simulink model "Kirov_physics"  (R2024b)
settings: Solver=FixedStepDiscrete  StartTime=0.0  StopTime=inf  FixedStep=dt  RelTol=1e-3
undefined symbols (not defined in the file): accel_O, airspeed_bp, alpha_B, alpha_bp, alphaFull, alphaOff, b, battery_capacity_bp, battery_current_bp, battery_initial_capacity_mAh, battery_voltage_table, beta_bp, betaFull, betaOff, brake, brakes, c, channels, CLa, Clb, Clp, CLq, Clr, Cma, Cmq, Cnb, Cnp, Cnr, current_table, DiscIntNeverNeededParam, dt, ELEV_bp, elevator, f, flap, flaps, FLAPS_bp, gear, heightFadeStart, heightOff, hgt_0, Inertia_body, Inertia_load, kInduced, L_aileron, L_throttle, LAILE_bp, lat_0, lon_0, M_aile, M_body, M_elev, M_flap, M_front_gear, M_load, M_main_gear, M_prop, M_rudd, M_spoiler, minWingHeight ... (+36)
libraries: sm_lib x673, simulink x58, nesl_utility x51, simulink_extras x24, uavmavlinklib x12, instrumentlib x4, vrlib x3, aerolibfltsims x3, sharedtransform x3, eeGeneralControl x2, aerolibutil x2, AP_Connector x2
(part 3 of 6)

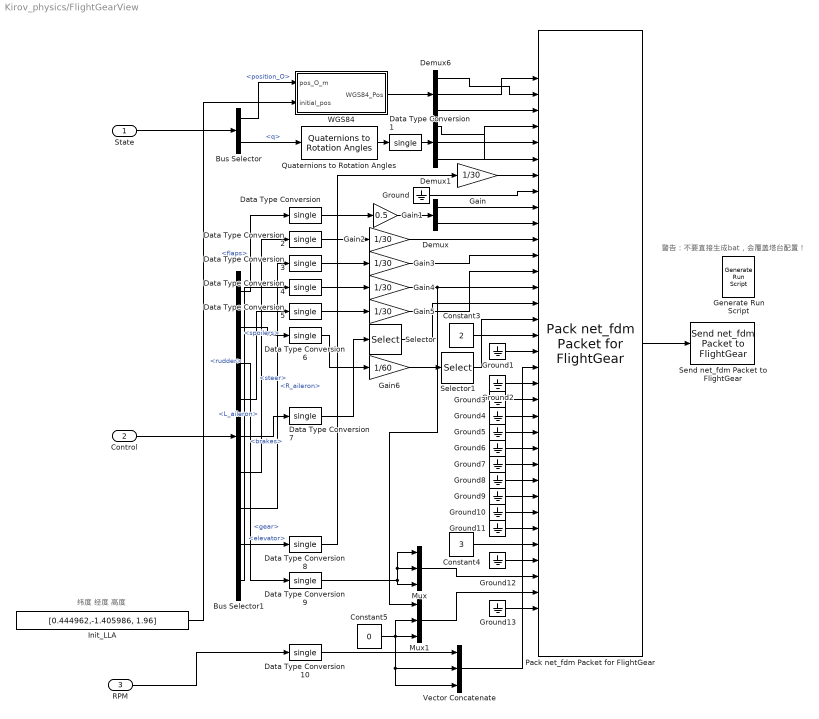
== system Kirov_physics/FlightGearView ==
  note: 警告：不要直接生成bat，会覆盖塔台配置！
  note: 纬度 经度 高度
  State : Inport
  Control : Inport  Port=2
  RPM : Inport  Port=3
  Bus Selector : BusSelector  OutputSignals=position_O,q
  Bus Selector1 : BusSelector  OutputSignals=flaps,spoilers,gear,steer,brakes,L_aileron,R_aileron,elevator,rudder
  Constant3 : Constant  Value=2  OutDataTypeStr=uint32
  Constant4 : Constant  Value=3  OutDataTypeStr=uint32
  Constant5 : Constant  Value=0  OutDataTypeStr=single
  Data Type Conversion{,1..10} (11 alike) : DataTypeConversion  OutDataTypeStr=single  SaturateOnIntegerOverflow=off  RndMeth=Floor
  Demux : Demux  Outputs=2
  Demux1 : Demux  Outputs=3
  Demux6 : Demux  Outputs=3
  Gain{,2..5} (5 alike) : Gain  Gain=1/30
  Gain1 : Gain  Gain=0.5
  Gain6 : Gain  Gain=1/60
  Generate Run Script : aerolibfltsims/Generate Run Script  Architecture=Win64  dataFlow=Send  GeometryModelName=Kirov  AirportId=X51  RunwayId=36  InitialAltitude=2  InitialHeading=0  OffsetDistance=0  OffsetAzimuth=0  InstallScenery=off  DisableShaders=off  OriginAddress=127.0.0.1  DestinationPort=5502  OriginPort=5505  LocalAddress=127.0.0.1  OutputFileName=runfg.bat  FlightGearBaseDirectory=E:\FlightGear 2024.1\
  Ground{,1..13} (14 alike) : Ground
  Init_LLA : Constant  Value=[0.444962,-1.405986, 1.96]  OutDataTypeStr=double
  Mux : Mux  Inputs=3
  Mux1 : Mux  Inputs=3
  Pack net_fdm Packet for FlightGear : aerolibfltsims/Pack net_fdm Packet for FlightGear  FlightGearVersion=v2019.1  ShowPositionAttitudeInputs=on  ShowVelocityAccelerationInputs=off  ShowControlSurfacePositionInputs=on  ShowEngineFuelInputs=on  ShowLandingGearInputs=on  ShowEnvironmentInputs=off  SampleTime=1/100  packetVersion=24
  Quaternions to Rotation Angles : sharedtransform/Quaternions to Rotation Angles  rotationOrder=ZYX  aMode=aMode
  Selector : Selector  InputPortWidth=2  IndexOptions=Index vector (dialog)  Indices=[1]  OutputSizes=1
  Selector1 : Selector  InputPortWidth=2  IndexOptions=Index vector (dialog)  Indices=[1]  OutputSizes=1
  Send net_fdm Packet to FlightGear : aerolibfltsims/Send net_fdm Packet to FlightGear  DestinationIpAddress=127.0.0.1  DestinationPort=5502  LocalIpPort=-1  varLen=off  SampleTime=1/100
  Vector Concatenate : Concatenate  NumInputs=3
  WGS84 : Subsystem
  wires:
  Data Type Conversion2/1 -> Gain2/1
  Quaternions to Rotation Angles/1 -> Data Type Conversion1/1
  State/1 -> Bus Selector/1
  Demux6/2 -> Pack net_fdm Packet for FlightGear/1
  Data Type Conversion1/1 -> Demux1/1
  Bus Selector1/7 -> Data Type Conversion3/1  "<R_aileron>"
  Data Type Conversion9/1 -> Mux/1, Mux/2, Mux/3
  Data Type Conversion5/1 -> Gain5/1
  Demux1/3 -> Pack net_fdm Packet for FlightGear/4
  Data Type Conversion4/1 -> Gain4/1
  Selector1/1 -> Pack net_fdm Packet for FlightGear/16
  Demux/1 -> Pack net_fdm Packet for FlightGear/9
  Gain4/1 -> Mux1/1, Pack net_fdm Packet for FlightGear/13
  Constant5/1 -> Mux1/3, Mux1/2, Vector Concatenate/2, Vector Concatenate/3
  Bus Selector1/4 -> Data Type Conversion5/1  "<steer>"
  Gain1/1 -> Demux/1
  Constant4/1 -> Pack net_fdm Packet for FlightGear/30
  Bus Selector1/8 -> Data Type Conversion8/1  "<elevator>"
  Ground/1 -> Pack net_fdm Packet for FlightGear/8
  Pack net_fdm Packet for FlightGear/1 -> Send net_fdm Packet to FlightGear/1
  Bus Selector1/9 -> Data Type Conversion4/1  "<rudder>"
  Demux1/2 -> Pack net_fdm Packet for FlightGear/5
  Vector Concatenate/1 -> Pack net_fdm Packet for FlightGear/19
  Constant3/1 -> Pack net_fdm Packet for FlightGear/17
  Ground6/1 -> Pack net_fdm Packet for FlightGear/24
  Ground11/1 -> Pack net_fdm Packet for FlightGear/29
  Ground7/1 -> Pack net_fdm Packet for FlightGear/25
  Mux1/1 -> Pack net_fdm Packet for FlightGear/33
  Ground9/1 -> Pack net_fdm Packet for FlightGear/27
  Ground8/1 -> Pack net_fdm Packet for FlightGear/26
  Bus Selector1/5 -> Data Type Conversion7/1  "<brakes>"
  Mux/1 -> Pack net_fdm Packet for FlightGear/32
  Bus Selector/1 -> WGS84/1(pos_O_m)  "<position_O>"
  Bus Selector/2 -> Quaternions to Rotation Angles/1  "<q>"
  Ground2/1 -> Pack net_fdm Packet for FlightGear/20
  WGS84/1(WGS84_Pos) -> Demux6/1
  Ground1/1 -> Pack net_fdm Packet for FlightGear/18
  Selector/1 -> Pack net_fdm Packet for FlightGear/15
  Data Type Conversion6/1 -> Gain6/1
  Gain3/1 -> Pack net_fdm Packet for FlightGear/12
  Ground5/1 -> Pack net_fdm Packet for FlightGear/23
  Bus Selector1/3 -> Data Type Conversion9/1  "<gear>"
  Ground3/1 -> Pack net_fdm Packet for FlightGear/21
  Bus Selector1/2 -> Data Type Conversion6/1  "<spoilers>"
  Demux/2 -> Pack net_fdm Packet for FlightGear/10
  Data Type Conversion3/1 -> Gain3/1
  Data Type Conversion7/1 -> Selector/1
  Ground4/1 -> Pack net_fdm Packet for FlightGear/22
  Ground12/1 -> Pack net_fdm Packet for FlightGear/31
  Data Type Conversion10/1 -> Vector Concatenate/1
  Gain5/1 -> Pack net_fdm Packet for FlightGear/14
  Gain2/1 -> Pack net_fdm Packet for FlightGear/11
  Ground10/1 -> Pack net_fdm Packet for FlightGear/28
  Ground13/1 -> Pack net_fdm Packet for FlightGear/34
  Demux1/1 -> Pack net_fdm Packet for FlightGear/6
  Data Type Conversion8/1 -> Gain/1
  Data Type Conversion/1 -> Gain1/1
  Bus Selector1/6 -> Data Type Conversion2/1  "<L_aileron>"
  Init_LLA/1 -> WGS84/2(initial_pos)
  Demux6/1 -> Pack net_fdm Packet for FlightGear/2
  Gain/1 -> Pack net_fdm Packet for FlightGear/7
  Bus Selector1/1 -> Data Type Conversion/1  "<flaps>"
  Demux6/3 -> Pack net_fdm Packet for FlightGear/3
  Control/1 -> Bus Selector1/1
  RPM/1 -> Data Type Conversion10/1
  Gain6/1 -> Selector1/1

== system Kirov_physics/Power ==
  Current : Inport
  Reset : ResetPort  DisableCoverage=on
  Battery_Voltage_LUT : Lookup_n-D  BreakpointsForDimension1=battery_current_bp  BreakpointsForDimension2=battery_capacity_bp  Table=battery_voltage_table  InterpMethod=Linear Lagrange  ExtrapMethod=Clip  InternalRulePriority=Speed  RndMeth=Simplest
      settings: InputPortMap=u0,u1
  Constant : Constant  Value=0
  Current_Limits : Saturate  UpperLimit=battery_current_bp(end)  LowerLimit=0
  Current_to_mAh_per_s : Gain  Gain=1/3.6
  Discharged_Capacity : DiscreteIntegrator  gainval=1  InitialCondition=battery_initial_capacity_mAh  SampleTime=-1  LimitOutput=on  UpperSaturationLimit=battery_capacity_bp(end)  LowerSaturationLimit=0  ShowSaturationPort=on  ICPrevOutput=DiscIntNeverNeededParam  ICPrevScaledInput=DiscIntNeverNeededParam
  Sum of Elements : Sum  Inputs=+
  Switch : Switch  Criteria=u2 > Threshold  Threshold=0.5  SaturateOnIntegerOverflow=off  InputSameDT=off
  voltage : Outport
  wires:
  Battery_Voltage_LUT/1 -> Switch/3  "V_bat_V"
  Discharged_Capacity/1 -> Battery_Voltage_LUT/2  "Q_dis_mAh"
  Current_to_mAh_per_s/1 -> Discharged_Capacity/1
  Current_Limits/1 -> Current_to_mAh_per_s/1, Battery_Voltage_LUT/1
  Sum of Elements/1 -> Current_Limits/1  "I_bus_A"
  Current/1 -> Sum of Elements/1
  Discharged_Capacity/2 -> Switch/2  "Battery_End"
  Switch/1 -> voltage/1
  Constant/1 -> Switch/1

== system Kirov_physics/Referee ==
  state : Inport
  Add Constant : Bias  Bias=50  SaturateOnIntegerOverflow=off
  Bus Selector : BusSelector  OutputSignals=position_O
  Constant : Constant  Value=2
  Constant1 : Constant  Value=0
  Demux : Demux  Outputs=3
  Gain : Gain  Gain=-1
  Less Than : RelationalOperator  Operator=<  OutDataTypeStr=boolean  RndMeth=Simplest  InputSameDT=off
  Less Than1 : RelationalOperator  Operator=<  OutDataTypeStr=boolean  RndMeth=Simplest  InputSameDT=off
  Less Than2 : RelationalOperator  Operator=>  OutDataTypeStr=boolean  RndMeth=Simplest  InputSameDT=off
  MATLAB Function1 : MATLAB Function  TreatAsAtomicUnit=on
  Manual Switch : ManualSwitch  CurrentSetting=0
  OR : Logic  Operator=OR  AllPortsSameDT=off  OutDataTypeStr=boolean
  Resettable Subsystem : Subsystem  TreatAsAtomicUnit=on
  Safety_Line : Constant  Value=0.5
  Stop Simulation : Stop
  Terminator : Terminator
  wires:
  state/1 -> Bus Selector/1
  Bus Selector/1 -> Demux/1  "<position_O>"
  Demux/1 -> Less Than2/1, Less Than1/1
  Demux/2 -> Less Than/1
  Safety_Line/1 -> Less Than/2
  Demux/3 -> Terminator/1
  Less Than/1 -> MATLAB Function1/1(u)
  Constant/1 -> Add Constant/1
  Less Than1/1 -> OR/1
  Add Constant/1 -> Gain/1, Less Than2/2
  Gain/1 -> Less Than1/2
  Less Than2/1 -> OR/2
  OR/1 -> Resettable Subsystem/1(beep)
  MATLAB Function1/1(y) -> Manual Switch/1
  Manual Switch/1 -> Stop Simulation/1
  Constant1/1 -> Manual Switch/2

== system Kirov_physics/SendState ==
  State : Inport
  Ardupilot : Subsystem  VariantControl=Ardupilot
  Mavlink : Subsystem  VariantControl=Mavlink

== system Kirov_physics/Train_Counter ==
  reset : Inport
  Add2 : Sum
  Minus : Sum  Inputs=+-
  Saturation : Saturate  UpperLimit=1  LowerLimit=0
  Unit Delay2 : UnitDelay  SampleTime=-1  HasFrameUpgradeWarning=on
  Unit Delay3 : UnitDelay  SampleTime=-1  HasFrameUpgradeWarning=on
  count : Outport
  wires:
  Unit Delay3/1 -> Add2/2
  Add2/1 -> count/1, Unit Delay3/1
  Unit Delay2/1 -> Minus/2
  Minus/1 -> Saturation/1
  reset/1 -> Minus/1, Unit Delay2/1
  Saturation/1 -> Add2/1

== system Kirov_physics/wind_NED ==
  wind_ned : Inport
  Bus Assignment : BusAssignment  AssignedSignals=timestamp,V_wind_O
  Constant : Constant  Value=0  OutDataTypeStr=Bus: Environment
  timestamp : Subsystem  mask{sample_time=1000*dt}
      mask prompts: sample_time "sample time (ms)"
  Env : Outport
  wires:
  Bus Assignment/1 -> Env/1
  Constant/1 -> Bus Assignment/1
  wind_ned/1 -> Bus Assignment/3
  timestamp/1(timestamp_ms) -> Bus Assignment/2

== system Kirov_physics/Actuator/Subsystem1 ==
  in : Inport
  Delay : Delay  DelayLengthSource=Input port  InitialConditionSource=Input port
      settings: InputPortMap=u0,p1,p4
  Divide : Product  Inputs=*/
  Round : Rounding  Operator=ceil
  delay_s : Constant  Value=delay_s
  dt_s : Constant  Value=dt
  dynamic_rate_saturation : Subsystem
  rate_limit_1/s : Constant  Value=rate_limit_per_s
  out : Outport
  wires:
  Round/1 -> Delay/2
  Delay/1 -> dynamic_rate_saturation/1(control_in)
  dynamic_rate_saturation/1(control_out) -> out/1  "out"
  in/1 -> Delay/3, Delay/1
  Divide/1 -> Round/1
  delay_s/1 -> Divide/1
  rate_limit_1/s/1 -> dynamic_rate_saturation/2(rate)
  dt_s/1 -> Divide/2

== system Kirov_physics/Actuator/Subsystem2 ==
  in : Inport
  Delay : Delay  DelayLengthSource=Input port  InitialConditionSource=Input port
      settings: InputPortMap=u0,p1,p4
  Divide : Product  Inputs=*/
  Round : Rounding  Operator=ceil
  delay_s : Constant  Value=delay_s
  dt_s : Constant  Value=dt
  dynamic_rate_saturation : Subsystem
  rate_limit_1/s : Constant  Value=rate_limit_per_s
  out : Outport
  wires:
  dt_s/1 -> Divide/2
  rate_limit_1/s/1 -> dynamic_rate_saturation/2(rate)
  delay_s/1 -> Divide/1
  Divide/1 -> Round/1
  in/1 -> Delay/1, Delay/3
  dynamic_rate_saturation/1(control_out) -> out/1  "out"
  Delay/1 -> dynamic_rate_saturation/1(control_in)
  Round/1 -> Delay/2

== system Kirov_physics/Actuator/Subsystem3 ==
  in : Inport
  Delay : Delay  DelayLengthSource=Input port  InitialConditionSource=Input port
      settings: InputPortMap=u0,p1,p4
  Divide : Product  Inputs=*/
  Round : Rounding  Operator=ceil
  delay_s : Constant  Value=delay_s
  dt_s : Constant  Value=dt
  dynamic_rate_saturation : Subsystem
  rate_limit_1/s : Constant  Value=rate_limit_per_s
  out : Outport
  wires:
  Round/1 -> Delay/2
  Delay/1 -> dynamic_rate_saturation/1(control_in)
  dynamic_rate_saturation/1(control_out) -> out/1  "out"
  in/1 -> Delay/3, Delay/1
  Divide/1 -> Round/1
  delay_s/1 -> Divide/1
  rate_limit_1/s/1 -> dynamic_rate_saturation/2(rate)
  dt_s/1 -> Divide/2

== system Kirov_physics/Actuator/Subsystem4 ==
  in : Inport
  Delay : Delay  DelayLengthSource=Input port  InitialConditionSource=Input port
      settings: InputPortMap=u0,p1,p4
  Divide : Product  Inputs=*/
  Round : Rounding  Operator=ceil
  delay_s : Constant  Value=delay_s
  dt_s : Constant  Value=dt
  dynamic_rate_saturation : Subsystem
  rate_limit_1/s : Constant  Value=rate_limit_per_s
  out : Outport
  wires:
  dt_s/1 -> Divide/2
  rate_limit_1/s/1 -> dynamic_rate_saturation/2(rate)
  delay_s/1 -> Divide/1
  Divide/1 -> Round/1
  in/1 -> Delay/1, Delay/3
  dynamic_rate_saturation/1(control_out) -> out/1  "out"
  Delay/1 -> dynamic_rate_saturation/1(control_in)
  Round/1 -> Delay/2

== system Kirov_physics/Actuator/Subsystem5 ==
  in : Inport
  Delay : Delay  DelayLengthSource=Input port  InitialConditionSource=Input port
      settings: InputPortMap=u0,p1,p4
  Divide : Product  Inputs=*/
  Round : Rounding  Operator=ceil
  delay_s : Constant  Value=delay_s
  dt_s : Constant  Value=dt
  dynamic_rate_saturation : Subsystem
  rate_limit_1/s : Constant  Value=rate_limit_per_s
  out : Outport
  wires:
  Round/1 -> Delay/2
  Delay/1 -> dynamic_rate_saturation/1(control_in)
  dynamic_rate_saturation/1(control_out) -> out/1  "out"
  in/1 -> Delay/3, Delay/1
  Divide/1 -> Round/1
  delay_s/1 -> Divide/1
  rate_limit_1/s/1 -> dynamic_rate_saturation/2(rate)
  dt_s/1 -> Divide/2

== system Kirov_physics/Actuator/Subsystem6 ==
  in : Inport
  Delay : Delay  DelayLengthSource=Input port  InitialConditionSource=Input port
      settings: InputPortMap=u0,p1,p4
  Divide : Product  Inputs=*/
  Round : Rounding  Operator=ceil
  delay_s : Constant  Value=delay_s
  dt_s : Constant  Value=dt
  dynamic_rate_saturation : Subsystem
  rate_limit_1/s : Constant  Value=rate_limit_per_s
  out : Outport
  wires:
  dt_s/1 -> Divide/2
  rate_limit_1/s/1 -> dynamic_rate_saturation/2(rate)
  delay_s/1 -> Divide/1
  Divide/1 -> Round/1
  in/1 -> Delay/1, Delay/3
  dynamic_rate_saturation/1(control_out) -> out/1  "out"
  Delay/1 -> dynamic_rate_saturation/1(control_in)
  Round/1 -> Delay/2

== system Kirov_physics/Actuator/Subsystem7 ==
  in : Inport
  Delay : Delay  DelayLengthSource=Input port  InitialConditionSource=Input port
      settings: InputPortMap=u0,p1,p4
  Divide : Product  Inputs=*/
  Round : Rounding  Operator=ceil
  delay_s : Constant  Value=delay_s
  dt_s : Constant  Value=dt
  dynamic_rate_saturation : Subsystem
  rate_limit_1/s : Constant  Value=rate_limit_per_s
  out : Outport
  wires:
  Round/1 -> Delay/2
  Delay/1 -> dynamic_rate_saturation/1(control_in)
  dynamic_rate_saturation/1(control_out) -> out/1  "out"
  in/1 -> Delay/3, Delay/1
  Divide/1 -> Round/1
  delay_s/1 -> Divide/1
  rate_limit_1/s/1 -> dynamic_rate_saturation/2(rate)
  dt_s/1 -> Divide/2

== system Kirov_physics/Actuator/Subsystem8 ==
  in : Inport
  Delay : Delay  DelayLengthSource=Input port  InitialConditionSource=Input port
      settings: InputPortMap=u0,p1,p4
  Divide : Product  Inputs=*/
  Round : Rounding  Operator=ceil
  delay_s : Constant  Value=delay_s
  dt_s : Constant  Value=dt
  dynamic_rate_saturation : Subsystem
  rate_limit_1/s : Constant  Value=rate_limit_per_s
  out : Outport
  wires:
  dt_s/1 -> Divide/2
  rate_limit_1/s/1 -> dynamic_rate_saturation/2(rate)
  delay_s/1 -> Divide/1
  Divide/1 -> Round/1
  in/1 -> Delay/1, Delay/3
  dynamic_rate_saturation/1(control_out) -> out/1  "out"
  Delay/1 -> dynamic_rate_saturation/1(control_in)
  Round/1 -> Delay/2

== system Kirov_physics/Actuator/timestamp ==
  Constant : Constant  Value=sample_time
  Data Type Conversion : DataTypeConversion  OutDataTypeStr=uint32  SaturateOnIntegerOverflow=off  RndMeth=Floor
  Discrete-Time Integrator : DiscreteIntegrator  IntegratorMethod=Accumulation: Forward Euler  SampleTime=-1  ICPrevOutput=DiscIntNeverNeededParam  ICPrevScaledInput=DiscIntNeverNeededParam
  timestamp_ms : Outport  VectorParamsAs1DForOutWhenUnconnected=off
  wires:
  Discrete-Time Integrator/1 -> Data Type Conversion/1
  Constant/1 -> Discrete-Time Integrator/1
  Data Type Conversion/1 -> timestamp_ms/1

== system Kirov_physics/Aerodynamics/GroundEffectCorrection ==
  fmBaseBody : Inport
  aeroAnglesDeg : Inport  Port=2
  positionO : Inport  Port=3
  refQ : Inport  Port=4
  ApplyGroundEffect : Subsystem
  GE_Enable : Constant
  fmBaseBodyGE : Outport
  wires:
  fmBaseBody/1 -> ApplyGroundEffect/1(fmBaseBody)
  aeroAnglesDeg/1 -> ApplyGroundEffect/2(aeroAnglesDeg)
  positionO/1 -> ApplyGroundEffect/3(positionO)
  GE_Enable/1 -> ApplyGroundEffect/4(GE_Enable)
  refQ/1 -> ApplyGroundEffect/5(refQ)
  ApplyGroundEffect/1(fmBaseBodyGE) -> fmBaseBodyGE/1

== system Kirov_physics/Aerodynamics/Wind2Body ==
  F_M : Inport
  alpha_beta : Inport  Port=2
  MATLAB Function : MATLAB Function  TreatAsAtomicUnit=on
  F_M_out : Outport
  wires:
  F_M/1 -> MATLAB Function/1(fmWind)
  alpha_beta/1 -> MATLAB Function/2(aeroAnglesDeg)
  MATLAB Function/1(fmBody) -> F_M_out/1

== system Kirov_physics/Aerodynamics/h2rho ==
  P_O : Inport
  COESA Atmosphere Model : aerolibatmos2/COESA Atmosphere Model  units=Metric (MKS)  spec=1976 COESA-extended U.S. Standard Atmosphere  model=Profile  profile_var=High temperature  profile_percent=1%  profile_alt=5 km (16404 ft)  envelope_var=High temperature  envelope_percent=1%  action=Warning
  Gain : Gain  Gain=-1
  Saturation : Saturate  UpperLimit=inf  LowerLimit=0
  Selector : Selector  InputPortWidth=3  IndexOptions=Index vector (dialog)  Indices=[3]  OutputSizes=1
  Signal Specification4 : SignalSpecification  OutDataTypeStr=double
  Terminator : Terminator
  Terminator1 : Terminator
  Terminator2 : Terminator
  rho : Outport
  wires:
  COESA Atmosphere Model/3 -> Terminator/1
  COESA Atmosphere Model/2 -> Terminator2/1
  Selector/1 -> Gain/1
  Gain/1 -> Saturation/1
  COESA Atmosphere Model/1 -> Terminator1/1
  Saturation/1 -> COESA Atmosphere Model/1
  Signal Specification4/1 -> rho/1
  P_O/1 -> Selector/1
  COESA Atmosphere Model/4 -> Signal Specification4/1

== system Kirov_physics/Aerodynamics/propulsion ==
  L_THRO : Inport
  R_THRO : Inport  Port=2
  voltage : Inport  Port=3
  Vx : Inport  Port=4
  Add : Sum
  Add1 : Sum
  Add2 : Sum
  Constant : Constant  Value=0
  Constant1 : Constant  Value=0
  Gain : Gain  Gain=-1
  Gain1 : Gain  Gain=0.8
  Gain2 : Gain  Gain=-0.8
  L_propeller : Subsystem
  Mux : Mux  Inputs=2
  Mux1 : Mux  Inputs=2
  R_propeller : Subsystem
  Saturation : Saturate  UpperLimit=12.6  LowerLimit=8
  Switch : Switch  Criteria=u2 > Threshold  Threshold=1  SaturateOnIntegerOverflow=off  InputSameDT=off
  Switch1 : Switch  Criteria=u2 > Threshold  Threshold=1  SaturateOnIntegerOverflow=off  InputSameDT=off
  Vector Concatenate : Concatenate  NumInputs=6
  F_M : Outport
  RPM : Outport  Port=2
  Current : Outport  Port=3
  wires:
  L_THRO/1 -> Switch1/1
  voltage/1 -> Switch1/2, Switch/2, Saturation/1
  Vx/1 -> R_propeller/3(Vx), L_propeller/3(Vx)
  Switch/1 -> R_propeller/1(throttle)
  R_propeller/3(rpm) -> Mux/2
  L_propeller/3(rpm) -> Mux/1
  Add/1 -> Vector Concatenate/1  "Thrust"
  L_propeller/1(thrust) -> Add/1, Gain1/1
  R_propeller/1(thrust) -> Add/2, Gain2/1
  Constant/1 -> Vector Concatenate/5, Vector Concatenate/3, Vector Concatenate/2
  L_propeller/2(torque) -> Gain/1
  Add1/1 -> Vector Concatenate/4
  Gain/1 -> Add1/1
  R_propeller/2(torque) -> Add1/2
  Gain1/1 -> Add2/1
  Gain2/1 -> Add2/2
  Add2/1 -> Vector Concatenate/6
  L_propeller/4(current) -> Mux1/1
  R_propeller/4(current) -> Mux1/2
  Mux1/1 -> Current/1
  Saturation/1 -> R_propeller/2(voltage), L_propeller/2(voltage)
  Vector Concatenate/1 -> F_M/1
  Mux/1 -> RPM/1
  R_THRO/1 -> Switch/1
  Constant1/1 -> Switch/3, Switch1/3
  Switch1/1 -> L_propeller/1(throttle)

== system Kirov_physics/Control_Input/Ardupilot ==
  AP receive : AP_Connector/AP receive  SystemSampleTime=-1  VariantActivationTime=update diagram  AllowFlexibleInterface=on  Latency=0  AutoFrameSizeCalculation=off
      link override MATLAB Function: SystemSampleTime=dt
      settings: SourceProductName=AP Connector
  Add Constant : Bias  Bias=-1500  SaturateOnIntegerOverflow=off
  Add Constant5 : Bias  Bias=1  SaturateOnIntegerOverflow=off
  Add Constant6 : Bias  Bias=1  SaturateOnIntegerOverflow=off
  Add Constant7 : Bias  Bias=1  SaturateOnIntegerOverflow=off
  Bus Assignment1 : BusAssignment  AssignedSignals=timestamp,throttle,roll,pitch,yaw,gear,flap,brake,spoiler
  Constant4 : Constant  Value=0  OutDataTypeStr=Bus: RCin
  Data Type Conversion : DataTypeConversion  OutDataTypeStr=uint8  SaturateOnIntegerOverflow=off  RndMeth=Floor
  Data Type Conversion1 : DataTypeConversion  OutDataTypeStr=uint8  SaturateOnIntegerOverflow=off  RndMeth=Floor
  Data Type Conversion2 : DataTypeConversion  OutDataTypeStr=uint8  SaturateOnIntegerOverflow=off  RndMeth=Floor
  Data Type Conversion3 : DataTypeConversion  OutDataTypeStr=double  SaturateOnIntegerOverflow=off  RndMeth=Floor
  Demux1 : Demux  Outputs=8
  Floor2 : Rounding  Operator=round
  Floor3 : Rounding  Operator=round
  Gain : Gain  Gain=1/500
  Gain10 : Gain  Gain=0.5
  Gain13 : Gain  Gain=0.5
  Saturation : Saturate  UpperLimit=2000  LowerLimit=1000
  Selector : Selector  InputPortWidth=16  IndexOptions=Index vector (dialog)  Indices=[13,15,12,16,5,1,7,3]  OutputSizes=1
  Terminator : Terminator
  timestamp1 : Subsystem  mask{sample_time=1000*dt}
      mask prompts: sample_time "sample time (ms)"
  Control_Input : Outport
  wires:
  Demux1/1 -> Bus Assignment1/4
  Demux1/7 -> Add Constant5/1
  Add Constant5/1 -> Gain10/1
  Demux1/3 -> Bus Assignment1/3
  Data Type Conversion2/1 -> Bus Assignment1/7
  Data Type Conversion/1 -> Bus Assignment1/8
  Data Type Conversion1/1 -> Bus Assignment1/9
  Gain10/1 -> Floor2/1
  Demux1/2 -> Bus Assignment1/5
  Demux1/5 -> Add Constant7/1
  Constant4/1 -> Bus Assignment1/1
  Gain13/1 -> Floor3/1
  Demux1/6 -> Add Constant6/1
  Demux1/4 -> Bus Assignment1/6
  Floor3/1 -> Data Type Conversion2/1
  Add Constant7/1 -> Gain13/1
  Demux1/8 -> Bus Assignment1/10
  Add Constant6/1 -> Data Type Conversion/1
  Floor2/1 -> Data Type Conversion1/1
  timestamp1/1(timestamp_ms) -> Bus Assignment1/2
  Bus Assignment1/1 -> Control_Input/1
  AP receive/2 -> Terminator/1
  AP receive/1 -> Data Type Conversion3/1
  Data Type Conversion3/1 -> Saturation/1
  Add Constant/1 -> Gain/1
  Gain/1 -> Selector/1
  Saturation/1 -> Add Constant/1
  Selector/1 -> Demux1/1

== system Kirov_physics/Control_Input/Joystick ==
  Add Constant5 : Bias  Bias=1  SaturateOnIntegerOverflow=off
  Add Constant6 : Bias  Bias=1  SaturateOnIntegerOverflow=off
  Add Constant7 : Bias  Bias=1  SaturateOnIntegerOverflow=off
  Bus Assignment1 : BusAssignment  AssignedSignals=timestamp,throttle,roll,pitch,yaw,gear,flap,brake,spoiler
  Constant4 : Constant  Value=0  OutDataTypeStr=Bus: RCin
  Data Type Conversion : DataTypeConversion  OutDataTypeStr=uint8  SaturateOnIntegerOverflow=off  RndMeth=Floor
  Data Type Conversion1 : DataTypeConversion  OutDataTypeStr=uint8  SaturateOnIntegerOverflow=off  RndMeth=Floor
  Data Type Conversion2 : DataTypeConversion  OutDataTypeStr=uint8  SaturateOnIntegerOverflow=off  RndMeth=Floor
  Demux1 : Demux  Outputs=8
  Floor2 : Rounding  Operator=round
  Floor3 : Rounding  Operator=round
  Gain10 : Gain  Gain=0.5
  Gain13 : Gain  Gain=0.5
  Joystick Input : vrlib/Joystick Input  joyid=1  adjustports=on  forcefeed=off
  Map : Selector  InputPortWidth=8  IndexOptions=Index vector (dialog)  Indices=[1 2 3 4 5 6 8 7]  OutputSizes=1
  Product : Product
  Rate Transition : RateTransition  Integrity=off  OutPortSampleTime=dt
  Reverse : Constant  Value=[1 1 1 1 1 1 1 1]
  Terminator : Terminator
  timestamp1 : Subsystem  mask{sample_time=1000*dt}
      mask prompts: sample_time "sample time (ms)"
  Control_Input : Outport
  wires:
  Demux1/1 -> Bus Assignment1/4
  Add Constant7/1 -> Gain13/1
  Gain10/1 -> Floor2/1
  Floor3/1 -> Data Type Conversion2/1
  Data Type Conversion/1 -> Bus Assignment1/8
  Demux1/3 -> Bus Assignment1/3
  Rate Transition/1 -> Map/1
  Map/1 -> Product/2
  Add Constant6/1 -> Data Type Conversion/1
  Demux1/2 -> Bus Assignment1/5
  Demux1/7 -> Add Constant5/1
  Demux1/6 -> Add Constant6/1
  Gain13/1 -> Floor3/1
  timestamp1/1(timestamp_ms) -> Bus Assignment1/2
  Data Type Conversion2/1 -> Bus Assignment1/7
  Joystick Input/1 -> Rate Transition/1
  Demux1/8 -> Bus Assignment1/10
  Add Constant5/1 -> Gain10/1
  Reverse/1 -> Product/1
  Product/1 -> Demux1/1
  Data Type Conversion1/1 -> Bus Assignment1/9
  Bus Assignment1/1 -> Control_Input/1
  Floor2/1 -> Data Type Conversion1/1
  Demux1/4 -> Bus Assignment1/6
  Joystick Input/2 -> Terminator/1
  Demux1/5 -> Add Constant7/1
  Constant4/1 -> Bus Assignment1/1

== system Kirov_physics/Control_Input/None ==
  Bus Assignment : BusAssignment  AssignedSignals=gear
  Constant1 : Constant  Value=0  OutDataTypeStr=Bus: RCin
  Constant2 : Constant  OutDataTypeStr=uint8
  Control_Input : Outport
  wires:
  Constant2/1 -> Bus Assignment/2
  Constant1/1 -> Bus Assignment/1
  Bus Assignment/1 -> Control_Input/1
